simulink model "bioreactor_simple"  (R2025b)
settings: Solver=VariableStepAuto  StartTime=0.0  StopTime=100  RelTol=1e-3
values from neighbouring files (symbols this model uses):
  D0 = 0.202    [bioreactor_init.m]
  xss = transpose(x_ss)    [bioreactor_init.m]
settings Model: Creator=sam  LastModifiedBy=sam

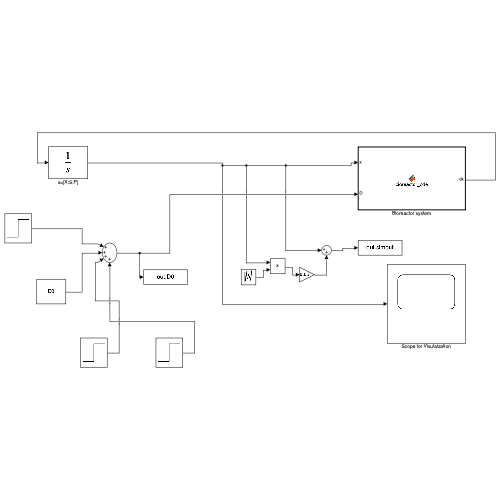
[thumbnail: Simulink's stored preview of the top-level diagram]
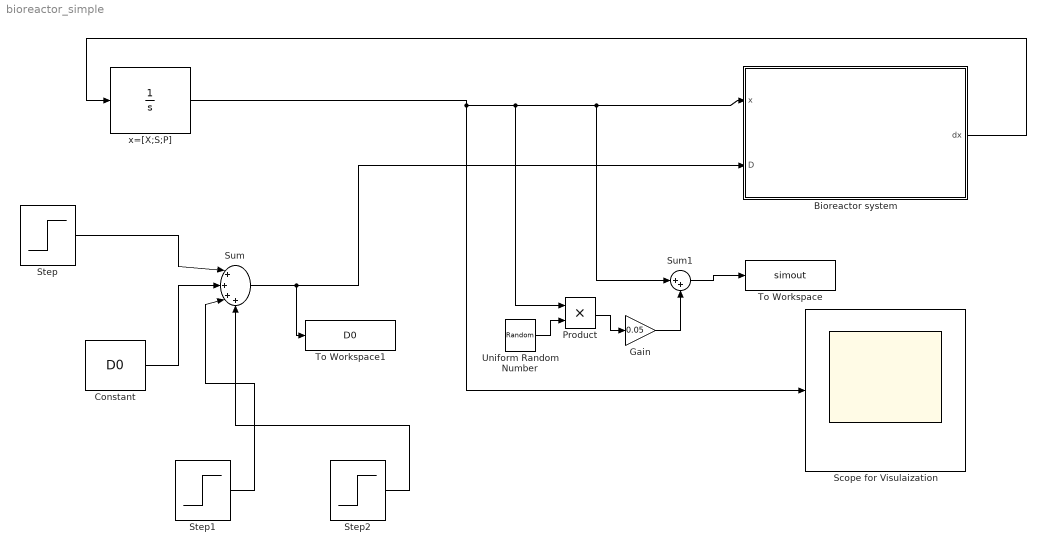
== system bioreactor_simple ==
  Bioreactor system : MATLAB Function  TreatAsAtomicUnit=on
  Constant : Constant  Value=D0
  Gain : Gain  Gain=0.05
  Product : Product
  Scope for Visulaization : Scope
      settings: ActiveDisplayYMinimum=-1068.1857600956014  ActiveDisplayYMaximum=495.4587046825859
  Step : Step  Time=10  After=0.05*D0  SampleTime=0
  Step1 : Step  Time=40  After=0.05*D0  SampleTime=0
  Step2 : Step  Time=70  After=0.05*D0  SampleTime=0
  Sum : Sum  Inputs=|++++
  Sum1 : Sum  Inputs=|++
  To Workspace : ToWorkspace  VariableName=simout  SaveFormat=Structure With Time  SampleTime=-1
  To Workspace1 : ToWorkspace  VariableName=D0  SaveFormat=Structure With Time  SampleTime=-1
  Uniform Random Number : UniformRandomNumber  SampleTime=0.1
  x=[X;S;P] : Integrator  InitialCondition=xss
  wires:
  Sum/1 -> To Workspace1/1, Bioreactor system/2(D)
  Bioreactor system/1(dx) -> x=[X;S;P]/1
  Constant/1 -> Sum/2
  Step/1 -> Sum/1
  Step1/1 -> Sum/3
  Step2/1 -> Sum/4
  x=[X;S;P]/1 -> Product/1, Sum1/1, Bioreactor system/1(x), Scope for Visulaization/1
  Sum1/1 -> To Workspace/1
  Uniform Random Number/1 -> Product/2
  Product/1 -> Gain/1
  Gain/1 -> Sum1/2

== matlab function bioreactor_simple/Bioreactor system ==
  data: x input; dx output; D input
function dx = bioreactor_ode(x, D)
    % Parameters (same as your MATLAB script)
    Yxs = 0.4;   % g/g
    beta = 0.2;  % h^(-1)
    Pm = 50;     % g/L
    Ki = 22;     % g/L
    alpha = 2.2; % g/g
    mum = 0.48;  % h^(-1)
    Km = 1.2;    % g/L
    Sf = 20;     % g/L
    % States
    X = x(1);
    S = x(2);
    P = x(3);
    % Specific growth rate mu(S,P)
    A  = Km + S + (S.^2)/Ki;
    mu = (mum * (1 - (P / Pm)) * S) / A;
    % State derivatives
    dx = zeros(3,1);
    dx(1) = -D * X + mu * X;
    dx(2) =  D * (Sf - S) - (1 / Yxs) * mu * X;
    dx(3) = -D * P + (alpha * mu + beta) * X;
end
